simulink model "MdlCtrl_qLPVMPCtower"  (R2023a)
settings: Solver=FixedStepAuto  StartTime=0.0  StopTime=10.0  FixedStep=DT  RelTol=1e-3
undefined symbols (not defined in the file or in its folder): beta, controlValue, Cq, Ct, DTc, fcOmegaCtrl, fcOmegaStatesCtrl, fcTowerCtrl, kVeFiltCtrl, lambda, Lin_points, n_h, omegabar, pMPC, qLPVMPC_RefLUT, qMPC, rMPC, Rotor_Lambda, towerSignCtrl, wecs, Xk07, xk07
settings Model: DataDictionary=DD_Mdl1.sldd  Creator=ditt_aj  LastModifiedBy=jdi
settings SolverCC: ZeroCrossControl=DisableAll  AlgebraicLoopSolver=TrustRegion  AutoInsertRateTranBlk=on
settings DataIOCC: SaveOutput=off  SaveTime=off
settings DebuggingCC: UnconnectedInputMsg=warning  UnconnectedOutputMsg=warning  UnconnectedLineMsg=warning
settings ModelReferenceCC: EnableRefExpFcnMdlSchedulingChecks=on
settings RTWCC: DLArmComputeVersion=19.05
settings GRTTargetCC: CombineOutputUpdateFcns=off  MatFileLogging=off

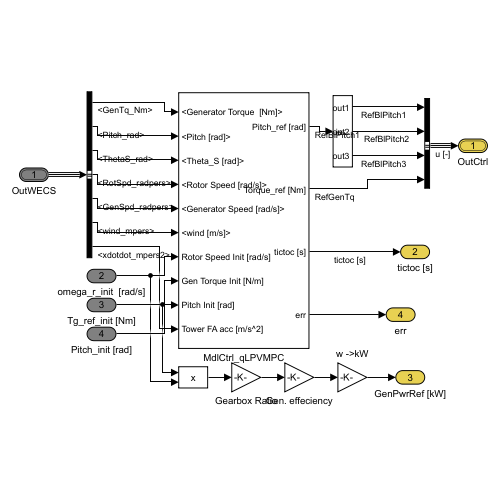
[thumbnail: Simulink's stored preview of the top-level diagram]
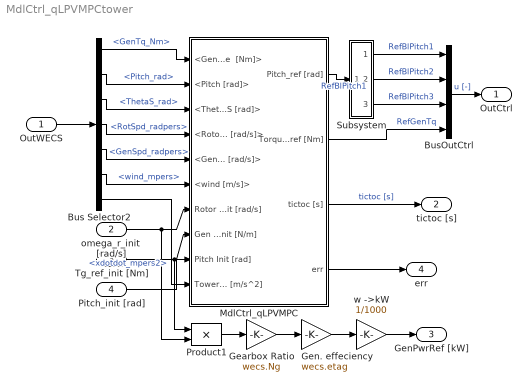
== system MdlCtrl_qLPVMPCtower ==
  OutWECS : Inport  OutDataTypeStr=Bus: slBus1  SampleTime=DTc
  omega_r_init  [rad/s] : Inport  Port=2  SampleTime=DTc
  Tg_ref_init [Nm] : Inport  Port=3  SampleTime=DTc
  Pitch_init [rad] : Inport  Port=4  SampleTime=DTc
  Bus Selector2 : BusSelector  OutputSignals=GenTq_Nm,Pitch_rad,ThetaS_rad,RotSpd_radpers,GenSpd_radpers,wind_mpers,xdotdot_mpers2
  BusOutCtrl : BusCreator  Inputs=4  OutDataTypeStr=Bus: slBus2
  Gearbox Ratio : Gain  Gain=wecs.Ng
  Gen. effeciency : Gain  Gain=wecs.etag
  MdlCtrl_qLPVMPC : Subsystem
  Product1 : Product  RndMeth=Zero
  Subsystem : Subsystem
  w ->kW : Gain  Gain=1/1000
  OutCtrl : Outport  OutDataTypeStr=Bus: slBus2  VectorParamsAs1DForOutWhenUnconnected=off
  tictoc [s] : Outport  Port=2
  GenPwrRef [kW] : Outport  Port=3
  err : Outport  Port=4
  wires:
  omega_r_init  [rad/s]/1 -> Product1/2, MdlCtrl_qLPVMPC/7(Rotor Speed Init [rad/s])
  Bus Selector2/6 -> MdlCtrl_qLPVMPC/6(<wind [m/s]>)  "<wind_mpers>"
  Bus Selector2/1 -> MdlCtrl_qLPVMPC/1(<Generator Torque  [Nm]>)  "<GenTq_Nm>"
  Bus Selector2/4 -> MdlCtrl_qLPVMPC/4(<Rotor Speed [rad/s]>)  "<RotSpd_radpers>"
  Bus Selector2/5 -> MdlCtrl_qLPVMPC/5(<Generator Speed [rad/s]>)  "<GenSpd_radpers>"
  Tg_ref_init [Nm]/1 -> Product1/1, MdlCtrl_qLPVMPC/8(Gen Torque Init [N/m])
  Pitch_init [rad]/1 -> MdlCtrl_qLPVMPC/9(Pitch Init [rad])
  Bus Selector2/3 -> MdlCtrl_qLPVMPC/3(<Theta_S [rad]>)  "<ThetaS_rad>"
  MdlCtrl_qLPVMPC/3(tictoc [s]) -> tictoc [s]/1  "tictoc [s]"
  Product1/1 -> Gearbox Ratio/1
  Gearbox Ratio/1 -> Gen. effeciency/1
  Gen. effeciency/1 -> w ->kW/1
  w ->kW/1 -> GenPwrRef [kW]/1
  OutWECS/1 -> Bus Selector2/1
  Bus Selector2/2 -> MdlCtrl_qLPVMPC/2(<Pitch [rad]>)  "<Pitch_rad>"
  Subsystem/2(out2) -> BusOutCtrl/2  "RefBlPitch2"
  BusOutCtrl/1 -> OutCtrl/1  "u [-]"
  Subsystem/1(out1) -> BusOutCtrl/1  "RefBlPitch1"
  Subsystem/3(out3) -> BusOutCtrl/3  "RefBlPitch3"
  MdlCtrl_qLPVMPC/1(Pitch_ref [rad]) -> Subsystem/1(in)  "RefBlPitch1"
  MdlCtrl_qLPVMPC/2(Torque_ref [Nm]) -> BusOutCtrl/4  "RefGenTq"
  MdlCtrl_qLPVMPC/4(err) -> err/1
  Bus Selector2/7 -> MdlCtrl_qLPVMPC/10(Tower FA acc [m/s^2])  "<xdotdot_mpers2>"

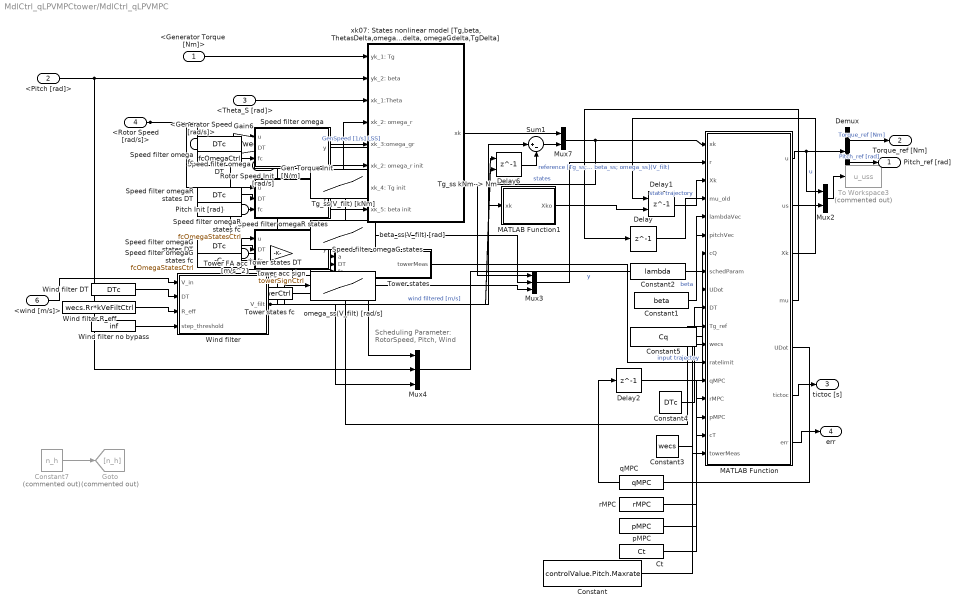
== system MdlCtrl_qLPVMPCtower/MdlCtrl_qLPVMPC ==
  note: Scheduling Parameter:
      | RotorSpeed, Pitch, Wind
  <Generator Torque  [Nm]> : Inport
  <Pitch [rad]> : Inport  Port=2
  <Theta_S [rad]> : Inport  Port=3
  <Rotor Speed [rad/s]> : Inport  Port=4
  <Generator Speed [rad/s]> : Inport  Port=5
  <wind [m/s]> : Inport  Port=6
  Rotor Speed Init [rad/s] : Inport  Port=7
  Gen Torque Init [N/m] : Inport  Port=8
  Pitch Init [rad] : Inport  Port=9
  Tower FA acc [m/s^2] : Inport  Port=10
  Constant : Constant  Value=controlValue.Pitch.Maxrate
  Constant1 : Constant  Value=beta
  Constant2 : Constant  Value=lambda
  Constant3 : Constant  Value=wecs  OutDataTypeStr=Bus: wecsBus
  Constant4 : Constant  Value=DTc
  Constant5 : Constant  Value=Cq
  Constant7 : Constant  Commented=on  Value=n_h
  Ct : Constant  Value=Ct
  Delay : Delay  DelayLength=1  InitialCondition=zeros(160,1)
  Delay1 : Delay  DelayLength=1  InitialConditionSource=Input port  InitialCondition=Xk07
      settings: InputPortMap=u0,p4
  Delay2 : Delay  DelayLength=1  InitialCondition=zeros(n_h*2,1)
  Delay6 : Delay  DelayLength=1  InitialConditionSource=Input port  InitialCondition=[0, Lin_points.Torque(1)]
      settings: InputPortMap=u0,p4
  Demux : Demux  Outputs=2
  Gain6 : Gain  Gain=1/wecs.Ng
  Goto : Goto  Commented=on  GotoTag=n_h
  MATLAB Function : MATLAB Function  TreatAsAtomicUnit=on
  MATLAB Function1 : MATLAB Function  TreatAsAtomicUnit=on
  Mux2 : Mux  Inputs=2
  Mux3 : Mux  Inputs=3
  Mux4 : Mux  Inputs=3
  Mux7 : Mux  Inputs=2
  Speed filter omega : MATLAB Function  TreatAsAtomicUnit=on
  Speed filter omega DT : Constant  Value=DTc
  Speed filter omega fc : Constant  Value=fcOmegaCtrl
  Speed filter omegaG states : MATLAB Function  TreatAsAtomicUnit=on
  Speed filter omegaG states DT : Constant  Value=DTc
  Speed filter omegaG states fc : Constant  Value=fcOmegaStatesCtrl
  Speed filter omegaR states : MATLAB Function  TreatAsAtomicUnit=on
  Speed filter omegaR states DT : Constant  Value=DTc
  Speed filter omegaR states fc : Constant  Value=fcOmegaStatesCtrl
  Sum1 : Sum  Inputs=|+-
  "Tg_ss kNm -> Nm" : Gain  Gain=1000
  Tg_ss(V_filt) [kNm] : Lookup_n-D  NumberOfTableDimensions=1  BreakpointsForDimension1=qLPVMPC_RefLUT.V  BreakpointsForDimension2=Rotor_Lambda  Table=qLPVMPC_RefLUT.Torque  InternalRulePriority=Speed  RndMeth=Simplest
  To Workspace3 : ToWorkspace  Commented=on  VariableName=u_uss  SampleTime=-1
      settings: Save2DSignal=2-D array (concatenate along first dimension)
  Tower acc sign : Gain  Gain=towerSignCtrl
  Tower states : MATLAB Function  TreatAsAtomicUnit=on
  Tower states DT : Constant  Value=DTc
  Tower states fc : Constant  Value=fcTowerCtrl
  Wind filter : MATLAB Function  TreatAsAtomicUnit=on
  Wind filter DT : Constant  Value=DTc
  Wind filter R_eff : Constant  Value=wecs.Rr*kVeFiltCtrl
  Wind filter no bypass : Constant  Value=inf
  beta_ss(V_filt) [rad] : Lookup_n-D  NumberOfTableDimensions=1  BreakpointsForDimension1=qLPVMPC_RefLUT.V  BreakpointsForDimension2=Rotor_Lambda  Table=qLPVMPC_RefLUT.Pitch  InternalRulePriority=Speed  RndMeth=Simplest
  omega_ss(V_filt) [rad/s] : Lookup_n-D  NumberOfTableDimensions=1  BreakpointsForDimension1=qLPVMPC_RefLUT.V  BreakpointsForDimension2=Rotor_Lambda  Table=qLPVMPC_RefLUT.RSpeed  InternalRulePriority=Speed  RndMeth=Simplest
  pMPC : Constant  Value=pMPC
  qMPC : Constant  Value=qMPC
  rMPC : Constant  Value=rMPC
  "xk07: States nonlinear model [Tg,beta, ThetasDelta,omegaRdelta, omegaGdelta,TgDelta]" : Subsystem
  Pitch_ref [rad] : Outport
  Torque_ref [Nm] : Outport  Port=2
  tictoc [s] : Outport  Port=3
  err : Outport  Port=4
  wires:
  Mux4/1 -> MATLAB Function/8(schedParam)  "y"
  Pitch Init [rad]/1 -> "xk07: States nonlinear model [Tg,beta, ThetasDelta,omegaRdelta, omegaGdelta,TgDelta]"/8(xk_5: beta init)
  MATLAB Function/4(mu) -> Delay/1
  Constant5/1 -> MATLAB Function/7(cQ)
  Sum1/1 -> Mux7/2
  Demux/1 -> Torque_ref [Nm]/1  "Torque_ref [Nm]"
  Mux2/1 -> To Workspace3/1
  MATLAB Function/1(u) -> Mux2/1, Demux/1  "u"
  <Theta_S [rad]>/1 -> "xk07: States nonlinear model [Tg,beta, ThetasDelta,omegaRdelta, omegaGdelta,TgDelta]"/3(xk_1:Theta)
  <Generator Torque  [Nm]>/1 -> "xk07: States nonlinear model [Tg,beta, ThetasDelta,omegaRdelta, omegaGdelta,TgDelta]"/1(yk_1: Tg)
  Gain6/1 -> "xk07: States nonlinear model [Tg,beta, ThetasDelta,omegaRdelta, omegaGdelta,TgDelta]"/5("xk_3:omega_gr ")  "GenSpeed [1/s] LSS]"
  MATLAB Function/2(us) -> Mux2/2
  Mux3/1 -> MATLAB Function/2(r)  "reference [Tg_ss; beta_ss; omega_ss](V_filt)"
  Delay/1 -> MATLAB Function/4(mu_old)
  <Pitch [rad]>/1 -> Mux4/2, "xk07: States nonlinear model [Tg,beta, ThetasDelta,omegaRdelta, omegaGdelta,TgDelta]"/2(yk_2: beta)
  MATLAB Function/3(Xk) -> Delay1/1
  MATLAB Function/6(tictoc) -> tictoc [s]/1
  Delay2/1 -> MATLAB Function/9("UDot ")  "input trajectoy"
  Demux/2 -> Pitch_ref [rad]/1  "Pitch_ref [rad]"
  Rotor Speed Init [rad/s]/1 -> "xk07: States nonlinear model [Tg,beta, ThetasDelta,omegaRdelta, omegaGdelta,TgDelta]"/6(xk_2: omega_r init)
  MATLAB Function/5(UDot) -> Delay2/1
  Mux7/1 -> MATLAB Function1/1(xk), MATLAB Function/1(xk)  "states"
  Constant4/1 -> MATLAB Function/10(DT)
  Delay6/1 -> Sum1/2
  Delay1/1 -> MATLAB Function/3("Xk ")  "state trajectory"
  "xk07: States nonlinear model [Tg,beta, ThetasDelta,omegaRdelta, omegaGdelta,TgDelta]"/1(xk) -> Mux7/1
  Constant2/1 -> MATLAB Function/5(lambdaVec)
  Constant1/1 -> MATLAB Function/6(pitchVec)  "beta"
  MATLAB Function1/1(Xko) -> Delay1/2
  Gen Torque Init [N/m]/1 -> "xk07: States nonlinear model [Tg,beta, ThetasDelta,omegaRdelta, omegaGdelta,TgDelta]"/7(xk_4: Tg init), MATLAB Function/11(Tg_ref)
  MATLAB Function/7(err) -> err/1
  Constant3/1 -> MATLAB Function/12(wecs)
  Constant7/1 -> Goto/1
  Constant/1 -> MATLAB Function/13(ratelimit)
  Wind filter DT/1 -> Wind filter/2(DT)
  Wind filter R_eff/1 -> Wind filter/3(R_eff)
  Wind filter no bypass/1 -> Wind filter/4(step_threshold)
  Wind filter/1(V_filt) -> Sum1/1, Delay6/1, Delay6/2, Mux4/3, Tg_ss(V_filt) [kNm]/1, beta_ss(V_filt) [rad]/1, omega_ss(V_filt) [rad/s]/1  "wind filtered [m/s]"
  Tg_ss(V_filt) [kNm]/1 -> "Tg_ss kNm -> Nm"/1
  "Tg_ss kNm -> Nm"/1 -> Mux3/1
  beta_ss(V_filt) [rad]/1 -> Mux3/2
  <wind [m/s]>/1 -> Wind filter/1(V_in)
  omega_ss(V_filt) [rad/s]/1 -> Mux3/3
  qMPC/1 -> MATLAB Function/14(qMPC)
  rMPC/1 -> MATLAB Function/15(rMPC)
  pMPC/1 -> MATLAB Function/16(pMPC)
  Speed filter omega/1(y) -> Mux4/1
  Speed filter omega DT/1 -> Speed filter omega/2(DT)
  Speed filter omega fc/1 -> Speed filter omega/3(fc)
  <Rotor Speed [rad/s]>/1 -> Speed filter omega/1(u), Speed filter omegaR states/1(u)
  Speed filter omegaR states/1(y) -> "xk07: States nonlinear model [Tg,beta, ThetasDelta,omegaRdelta, omegaGdelta,TgDelta]"/4(xk_2: omega_r)
  Speed filter omegaR states DT/1 -> Speed filter omegaR states/2(DT)
  Speed filter omegaR states fc/1 -> Speed filter omegaR states/3(fc)
  <Generator Speed [rad/s]>/1 -> Speed filter omegaG states/1(u)
  Speed filter omegaG states/1(y) -> Gain6/1
  Speed filter omegaG states DT/1 -> Speed filter omegaG states/2(DT)
  Speed filter omegaG states fc/1 -> Speed filter omegaG states/3(fc)
  Tower states DT/1 -> Tower states/2(DT)
  Tower states fc/1 -> Tower states/3(fc)
  Ct/1 -> MATLAB Function/17(cT)
  Tower states/1(towerMeas) -> MATLAB Function/18(towerMeas)
  Tower FA acc [m/s^2]/1 -> Tower acc sign/1
  Tower acc sign/1 -> Tower states/1(a)

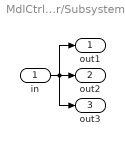
== system MdlCtrl_qLPVMPCtower/Subsystem ==
  in : Inport
  out1 : Outport
  out2 : Outport  Port=2
  out3 : Outport  Port=3
  wires:
  in/1 -> out1/1, out2/1, out3/1

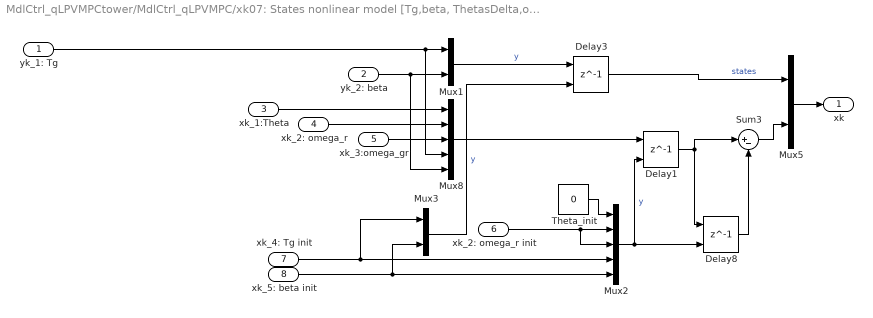
== system MdlCtrl_qLPVMPCtower/MdlCtrl_qLPVMPC/xk07: States nonlinear model [Tg,beta, ThetasDelta,omegaRdelta, omegaGdelta,TgDelta] ==
  yk_1: Tg : Inport
  yk_2: beta : Inport  Port=2
  xk_1:Theta : Inport  Port=3
  xk_2: omega_r : Inport  Port=4
  "xk_3:omega_gr " : Inport  Port=5
  xk_2: omega_r init : Inport  Port=6
  xk_4: Tg init : Inport  Port=7
  xk_5: beta init : Inport  Port=8
  Delay1 : Delay  DelayLength=1  InitialConditionSource=Input port  InitialCondition=[0,omegabar]
      settings: InputPortMap=u0,p4
  Delay3 : Delay  DelayLength=1  InitialConditionSource=Input port  InitialCondition=xk07
      settings: InputPortMap=u0,p4
  Delay8 : Delay  DelayLength=1  InitialConditionSource=Input port  InitialCondition=[0,omegabar]
      settings: InputPortMap=u0,p4
  Mux1 : Mux  Inputs=2
  Mux2 : Mux  Inputs=5
  Mux3 : Mux  Inputs=2
  Mux5 : Mux  Inputs=2
  Mux8 : Mux  Inputs=5
  Sum3 : Sum  Inputs=|+-
  Theta_init : Constant  Value=0
  xk : Outport  VectorParamsAs1DForOutWhenUnconnected=off
  wires:
  xk_4: Tg init/1 -> Mux3/1, Mux2/4
  xk_2: omega_r init/1 -> Mux2/2, Mux2/3
  Theta_init/1 -> Mux2/1
  xk_5: beta init/1 -> Mux3/2, Mux2/5
  xk_1:Theta/1 -> Mux8/1
  xk_2: omega_r/1 -> Mux8/2
  "xk_3:omega_gr "/1 -> Mux8/3
  Mux5/1 -> xk/1
  Mux2/1 -> Delay1/2, Delay8/2  "y"
  yk_2: beta/1 -> Mux1/2, Mux8/5
  Delay8/1 -> Sum3/2
  yk_1: Tg/1 -> Mux1/1, Mux8/4
  Sum3/1 -> Mux5/2
  Delay3/1 -> Mux5/1  "states"
  Mux1/1 -> Delay3/1  "y"
  Mux3/1 -> Delay3/2  "y"
  Mux8/1 -> Delay1/1
  Delay1/1 -> Sum3/1, Delay8/1

== matlab function MdlCtrl_qLPVMPCtower/MdlCtrl_qLPVMPC/Tower states ==
  data: a input; towerMeas output; DT input; fc input
function towerMeas = tower_states(a, DT, fc)
% Tower fore-aft velocity and displacement from the measured acceleration
% (leaky integration with corner frequency fc [Hz] against drift).
% towerMeas = [dx_t; dv_t; v_t]: increments over one sample and velocity
persistent v x
if isempty(v)
    v = 0;
    x = 0;
end
lam = exp(-2*pi*fc*DT);
vNew = lam*v + a*DT;
xNew = lam*x + vNew*DT;
towerMeas = [xNew - x; vNew - v; vNew];
v = vNew;
x = xNew;

== matlab function MdlCtrl_qLPVMPCtower/MdlCtrl_qLPVMPC/MATLAB Function1 ==
  data: xk input; Xko output
function Xko = fcnKron(xk)

Xko = kron(ones(40,1),[xk(1:2); 0; 0; xk(3:7); 0; 0; xk(8); 0; 0]); % rotor speed (set in qLPVMPC_WECS_beta), tower states
% and delayed input increments (14 augmented states)

== matlab function MdlCtrl_qLPVMPCtower/MdlCtrl_qLPVMPC/MATLAB Function ==
  settings: updateMethod=DISCRETE
  data: xk input; r input; u output; us output; Xk input; mu_old input; lambdaVec input; pitchVec input; cQ input; schedParam input; UDot input; DT input; Xk output; mu output; UDot output; tictoc output; Tg_ref input; err output; wecs input; ratelimit input; qMPC input; rMPC input; pMPC input; cT input; towerMeas input
function [u,us,Xk,mu,UDot,tictoc,err] = qLPVMPC_WECS_beta(xk,r, Xk,mu_old,lambdaVec,pitchVec,cQ,schedParam,UDot,DT,Tg_ref,wecs,ratelimit,qMPC,rMPC,pMPC,cT,towerMeas)
% MATLAB_Function calculates controller output u. It turns the QP into a
% linear complementarity problem (LCP) and solves it with Lemke's algorithm.
%
% Inputs: * r: reference
%         * xk: quasiLPV KF state estimates
%              with xk = [Tg,beta,dThetas,dOmegaR,dOmega_g,dTg,dBeta, dV]
%              (the measured rotor speed is added as state 3)
%         * Xk: Xko(= L*xk+S*U) delayed by one sample timestep
%         * mu_old: mu delayed by one sample timestep
%         * lambdaVec: lambda vector for cQ LUT
%         * pitchVec: pitch vector for cQ LUT
%         * cQ: torque coefficients LUT matrix
%         * schedParam: current values [omegaR, beta, V]
%         * qMPC, rMPC: state and input weights (stage cost x'Qx + u'Ru)
%         * pMPC: terminal weight factor (P = pMPC*Q)
%         * cT: thrust coefficient table (tower model)
%         * towerMeas: [dx_t; dv_t; v_t] from the tower acceleration
%         * U: U (from Xko = L*xk+S*U) delayed by one sample timestep
%
% Outputs: * u: controller output at current time step
%          * Xko: Future state trajectory (L*xk+S*U)
%          * U: Future input trajectory
%          * mu: Result Lemke's algorithm/LCP: M mu +q >=0, mu>=0, mu'(Mmu+q)=0
%          * us: xuss(end) from xuss = [eye(4)-Ass -Bss;[1 0 0 0] 0]\[Bss*d;1]
%          * tictoc: tic-toc result

% Pablo S.G. Cisneros, Herbert Werner, ICS TUHH

%#codegen
coder.extrinsic('tic');
coder.extrinsic('toc');
tictoc = 0;
tic
optimLemke = 1; % Solve QP as linear complementary problem or use quadprog

%% Init N, Q, R
N = 40;
q_ = reshape(qMPC, 1, []); % [Tg, beta, OmegaR, dThetaS, dOmegaR, dOmegaG, dTg, dBeta, dV, dU(k-1)], third: rotor speed tracking % last two: delayed input increments (unweighted) %[10^4 0.1 1 1 100 0.1 0]; %q_ = [100 1000 1 0.01 0]; 7.351e+02 1.000e+00 1.938e+09 1.625e+08 1.491e+08 1.657e+03
r_ = reshape(rMPC, 1, []); % [dTg, dBeta]
R_ = kron(eye(N),diag(r_)); %R_ = 1000*eye(N);
p = pMPC*q_; %P = 1000*diag(q_);

u_rate_upper = [20000 * DT; ratelimit * pi/180 * DT];% Upper rate limit per sample: torque 20 kNm/s, pitch 13 deg/s
u_rate_lower = - u_rate_upper; % Lower rate limit
Ulim = [repmat(-u_rate_lower ,N,1);repmat(u_rate_upper ,N,1)]; % rate constraints

Control_Pitch_Max = 90 /180 * pi;
Control_Pitch_Min = 0 /180 * pi;
Control_Torque_Limit = 47403;
Control_Torque_Min = 200;

% isBetaState = 0;
% nx = 4 + isBetaState; % number states plant: ThetaS,omegaR,omegaG,Tg
% ny = 2 + isBetaState; % number of outputs plant omegaG,Tg
nxA = 14; % augmented states: [Tg, beta, OmegaR, v_t, dThetaS, dOmegaR, dOmegaG, dTg, dBeta, dx_t, dv_t, dV, dTg_ref(k-1), dBeta_ref(k-1)]
nu = 2; % plant inputs: Tg_ref, beta_ref

% Plausible scheduling values (e.g. zero samples after a rate transition at the start)
schedParam(1) = min(max(schedParam(1), 0.3), 2); % rotor speed [rad/s]
schedParam(2) = min(max(schedParam(2), 0), Control_Pitch_Max); % pitch [rad]
schedParam(3) = min(max(schedParam(3), 3), 30); % wind speed [m/s]

%% Previous command and increment (actuator delay states)
persistent u_prev dU_prev
if isempty(u_prev)
    u_prev = [Tg_ref; schedParam(2)];
    dU_prev = [0; 0];
    Xk(3:nxA:end) = schedParam(1); % the initial trajectory contains no rotor speed
end
xkA = [xk(1:2); schedParam(1); towerMeas(3); xk(3:7); towerMeas(1:2); xk(8); dU_prev]; % measured rotor speed and tower states

%% Shift Xk
Xk(1:end-nxA) = Xk(nxA+1:end);
UDot(1:end-nu) = UDot(nu+1:end);
if any(~isfinite(Xk)) % invalid trajectory: restart it from the current state
    Xk = repmat(xkA, N, 1);
end
UDot(~isfinite(UDot)) = 0;
%Xk(1:nxA)

%% Calculate input u_dot_s = 0  and steady state x = r
us = [0;0]; %xuss(nxA+1:nxA+2); % xuss = [eye(size(Ass))-Ass -Bss;[1 0 0 0] 0] \ [Bss*d;reference];

iterations = 1; % omega_ref(Vest), Tg_ref(Vest)
refVec = zeros(nxA,1);
refVec(1:3) = r; % [Tg_ss; beta_ss; omega_ss]
ref = repmat(refVec,N,1); %ref = kron(ones(N,1),[r; 0; 0; 0;0]);

for i = 1:iterations
    [L,S,H,g] = HSqLd_WT_tower(N,q_,R_,p,xkA,Xk,DT,ref,us,lambdaVec,pitchVec,cQ,cT,schedParam,UDot,wecs);

    %% %%%%%%Turn QP into LCP and solve it%%%%%%%%%

    % Set actuator rate constraints
    Ac_ = [-eye(N*nu);eye(N*nu)]; 
    bc_ = - Ulim;

    if optimLemke == 1

        Hi = eye(size(H,1))/H;
        M = Ac_*Hi*Ac_';
        q = -Ac_*Hi*g - bc_;

        mu0 = mu_old;
        mu0(~isfinite(mu0)) = 0; % never warm-start from a failed solution
        [mu,err] = lemke(M,q,mu0);
        UDot = Hi*(Ac_'*mu-g);
        % UDot(isnan(UDot)) = 0; % This should never happen. If it does err = 1
    else

        H1 = (H+H')/2;
        onlyFiniteElemts = isnumeric( H1) && all(isfinite( H1(:)));
        if onlyFiniteElemts
            options1 = optimoptions('quadprog','Display','none', 'Algorithm','active-set');
            UDot = quadprog((H+H')/2,g, Ac_, -bc_,[], [],[],[], UDot,options1);
            err = 0;
        else
            err = 1;
        end
    end

    if any(~isfinite(UDot)) % treat a non-finite solution as solver failure
        err = 1;
    end

    %% %%%%%%%%%%%%%%%%%%%%%%%%%%%%%%%%%%%%%%%%%%%
    if err == 0 % should be zero, otherwise don't update
        Xk = L*xkA+S*UDot;
    else
        % Solver failed: use the unconstrained optimum clipped to the rate
        % limits and reset the warm start
        UDot = min(max(-(H\g), -Ulim(N*nu+1:end)), Ulim(N*nu+1:end));
        mu(:) = 0;
        UDot(~isfinite(UDot)) = 0;
        Xk = L*xkA+S*UDot;
    end
end

% Command = previous command + increment, so the rate limit applies to the
% actuator reference itself
u =  [ min(max(u_prev(1) + UDot(1), Control_Torque_Min),Control_Torque_Limit),... % torque
    min( max(u_prev(2) + UDot(2), Control_Pitch_Min),Control_Pitch_Max)]'; % pitch
dU_prev = u - u_prev; % increment actually applied (after limits)
u_prev = u;

tictoc = toc;

% For debugging
%%%%%%%%%%% Compute Hessian H, derivative g = dJk/dUk %%
% min Jk(Uk) s.t. h1(Uk) = 0, h2(Uk) < 0, at current estimate xl
% <=> min( x'H(xl)x + g(xl)x s.t. dh1(xl)x+h1(xl)=0, dh2(xl)x+h2(xl)< 0
% with
% Jk = (Lx+SUk-Xss)'Q(Lx+SUk-Xss) +(Uk-Uss)'R(Uk-Uss) + Psi
% dJk/dUk = 2S'Q (Lx+SUk-Xss) + 2R(Uk-Uss)
% diffX = Xk(1:(end - nxA)) - ref(1:(end -nxA));
% diffXEnd = Xk((end - nxA +1):end) - ref((end - nxA +1):end);
%
% % Q_ = kron(eye(N-1),diag(q_));
% % Qcomp = diffX' * Q_ * diffX;
% % Pcomp = diffXEnd' * diag(p)* diffXEnd;
% % Rcomp = U' * R_ * U;
%
% diffXMat = sum(reshape(diffX.^2, nxA, N-1),2);
% UMat = sum(reshape(UDot.^2, 2, N),2);
%
% Qcomp = diffXMat' .* q_;
% Pcomp = (diffXEnd') .^2  .* p;
% Rcomp = UMat' .* r_;

== matlab function MdlCtrl_qLPVMPCtower/MdlCtrl_qLPVMPC/Wind filter ==
  settings: updateMethod=DISCRETE
  data: V_in input; V_filt output; DT input; R_eff input; step_threshold input
function V_filt = wind_filter(V_in, DT, R_eff,step_threshold)
% SPATIAL_WIND_FILTER 
% Implements a discrete, velocity-dependent low-pass filter for rotor-effective 
% wind speed estimation with an automated threshold bypass for step changes.

    % Persistent variables retain their state between time-steps
    persistent V_filt_prev V_in_prev 
    
    % --- Step 1: Handle Simulation Initialization ---
    if isempty( V_filt_prev) 
        V_filt_prev    = V_in; % Initialize filter state to current wind
        V_in_prev      = V_in; % Initialize raw input tracking
    end
    
    % --- Step 2: Compute Raw Wind Acceleration (Step Detection) ---
    % Calculate the true absolute sample-to-sample difference of the RAW wind
    delta_V_raw = abs(V_in - V_in_prev);
    
    % --- Step 3: Compute Filter Coefficient or Bypass ---
    % Compare with wind step threshold, e.g., 0.5 m/s jump between steps of 0.008s
    
    if delta_V_raw > step_threshold
        % If a non-physical step change is detected, snap alpha wide open
        alpha = 1.0;
    else
        %Otherwise, use the physical velocity-dependent spatial filter
        %Ensure V_in is bound to prevent division by zero at startup
        V_bound = max(V_in, 0.1); 
        alpha = 1.0 - exp(- (DT * V_bound) / R_eff);
        
       % Spherically bound alpha to normal discrete operational limits [0, 1]
        alpha = max(min(alpha, 1.0), 0.0);
   end
    
    % --- Step 4: Run the Filter Difference Equation ---
    V_filt = V_filt_prev + alpha * (V_in - V_filt_prev);
    
    % --- Step 5: Save State Registers for Next Step ---
    V_filt_prev = V_filt;
    V_in_prev   = V_in;
end

== matlab function MdlCtrl_qLPVMPCtower/MdlCtrl_qLPVMPC/Speed filter omega ==
  data: u input; y output; DT input; fc input
function y = speed_filter(u, DT, fc)
% First-order low-pass filter of a measured speed, corner frequency fc [Hz] (Inf: no filter)
persistent yPrev
if isempty(yPrev)
    yPrev = u;
end
alpha = 1 - exp(-2*pi*fc*DT);
y = yPrev + alpha*(u - yPrev);
yPrev = y;

== matlab function MdlCtrl_qLPVMPCtower/MdlCtrl_qLPVMPC/Speed filter omegaR states ==
  data: u input; y output; DT input; fc input
function y = speed_filter(u, DT, fc)
% First-order low-pass filter of a measured speed, corner frequency fc [Hz] (Inf: no filter)
persistent yPrev
if isempty(yPrev)
    yPrev = u;
end
alpha = 1 - exp(-2*pi*fc*DT);
y = yPrev + alpha*(u - yPrev);
yPrev = y;

== matlab function MdlCtrl_qLPVMPCtower/MdlCtrl_qLPVMPC/Speed filter omegaG states ==
  data: u input; y output; DT input; fc input
function y = speed_filter(u, DT, fc)
% First-order low-pass filter of a measured speed, corner frequency fc [Hz] (Inf: no filter)
persistent yPrev
if isempty(yPrev)
    yPrev = u;
end
alpha = 1 - exp(-2*pi*fc*DT);
y = yPrev + alpha*(u - yPrev);
yPrev = y;
